simulink model "EdgeImpulse_YOLO_Simulink"  (R2023b)
settings: Solver=FixedStepDiscrete  StartTime=0  StopTime=0.20000000000000001  FixedStep=0.10000000000000001  RelTol=1e-3
InitFcn:
  | ei_sim_prepare('EdgeImpulse_YOLO_Simulink');
model workspace (MAT data in the model file):
  eiBuildInfo.buildKey = 'eb16cb243767a9c4559b'
  eiBuildInfo.height = 180
  eiBuildInfo.width = 180
  eiImageSequence = timeseries
  eiImageSequence.Name = 'unnamed'
  eiImageSequence.DataInfo = tsdata.datametadata
  eiImageSequence.DataInfo.Interpolation = tsdata.interpolation
  eiImageSequence.DataInfo.Interpolation.Fhandle : function handle (value not decoded)
  eiImageSequence.DataInfo.Interpolation.Name = 'zoh'
  eiImageSequence.TimeInfo = tsdata.timemetadata
  eiImageSequence.TimeInfo.Length = 3
  eiImageSequence.TimeInfo.DuplicateTimes = 0
  eiImageSequence.TimeInfo.Time_ = [0; 0.1; 0.2]
  eiImageSequence.TimeInfo.Initialized = 1
  eiImageSequence.QualityInfo = tsdata.qualmetadata
  eiImageSequence.Data_ = [0 0 0 0 0 0 0 0 0 0 0 0 ... (97200 elements, 180x180x3)]
  eiImageSequence.IsTimeFirst_ = 0
  eiNewImageSequence = timeseries
  eiNewImageSequence.Name = 'unnamed'
  eiNewImageSequence.DataInfo = tsdata.datametadata
  eiNewImageSequence.DataInfo.Interpolation = tsdata.interpolation
  eiNewImageSequence.DataInfo.Interpolation.Fhandle : function handle (value not decoded)
  eiNewImageSequence.DataInfo.Interpolation.Name = 'zoh'
  eiNewImageSequence.TimeInfo = tsdata.timemetadata
  eiNewImageSequence.TimeInfo.Length = 3
  eiNewImageSequence.TimeInfo.DuplicateTimes = 0
  eiNewImageSequence.TimeInfo.Time_ = [0; 0.1; 0.2]
  eiNewImageSequence.TimeInfo.Initialized = 1
  eiNewImageSequence.QualityInfo = tsdata.qualmetadata
  eiNewImageSequence.Data_ = [1; 0; 0]
settings Model: Creator=saray  LastModifiedBy=saray
settings SFSimCC: SimCustomInitializer="{ int32_t s=ei_sim_start(5.000000000e-01f,0u,4096u,0u,0); if(s<0) { char e[1024]; ei_get_last_error(e,1024); mexErrMsgIdAndTxt(\"EI:SimInit\",\"%s\",e); } }"  SimCustomTerminator=ei_sim_stop();  SimUserIncludeDirs="\"C:\\Ago-Dic26\\VSCode\\Edge_Impules\\Audrey_Lazara\\EdgeImpulse_MATLAB_Integration\\native\""  SimUserLibraries="\"C:\\Ago-Dic26\\VSCode\\Edge_Impules\\Audrey_Lazara\\EdgeImpulse_MATLAB_Integration\\build\\eb16cb243767a9c4559b\\cmake\\lib\\libei_inference_eb16cb243767a9c4559b.dll.a\""  SimTargetLang=C++
settings SFSimCC: SimCustomHeaderCode=|
  | #include "ei_wrapper.h"
  | #include "mex.h"

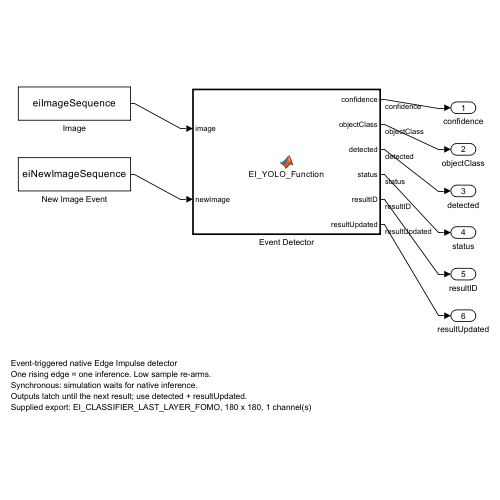
[thumbnail: Simulink's stored preview of the top-level diagram]
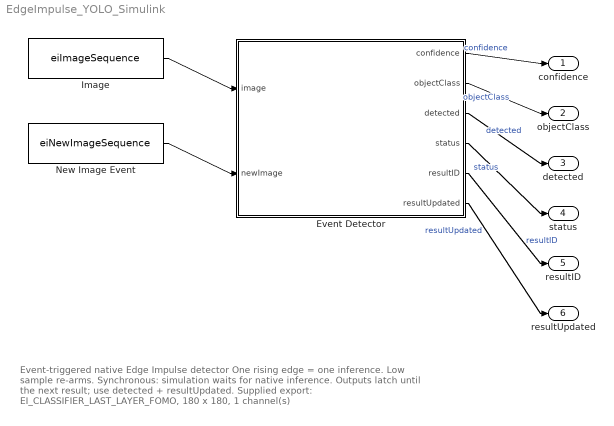
== system EdgeImpulse_YOLO_Simulink ==
  note: Event-triggered native Edge Impulse detector
      | One rising edge = one inference. Low sample re-arms.
      | Synchronous: simulation waits for native inference.
      | Outputs latch until the next result; use detected + resultUpdated.
      | Supplied export: EI_CLASSIFIER_LAST_LAYER_FOMO, 180 x 180, 1 channel(s)
  Event Detector : MATLAB Function  TreatAsAtomicUnit=on
  Image : FromWorkspace  VariableName=eiImageSequence  SampleTime=0.10000000000000001  Interpolate=off  OutputAfterFinalValue=Holding final value
  New Image Event : FromWorkspace  VariableName=eiNewImageSequence  SampleTime=0.10000000000000001  Interpolate=off  OutputAfterFinalValue=Holding final value
  confidence : Outport
  objectClass : Outport  Port=2
  detected : Outport  Port=3
  status : Outport  Port=4
  resultID : Outport  Port=5
  resultUpdated : Outport  Port=6
  wires:
  Image/1 -> Event Detector/1(image)
  New Image Event/1 -> Event Detector/2(newImage)
  Event Detector/1(confidence) -> confidence/1  "confidence"
  Event Detector/2(objectClass) -> objectClass/1  "objectClass"
  Event Detector/3(detected) -> detected/1  "detected"
  Event Detector/4(status) -> status/1  "status"
  Event Detector/5(resultID) -> resultID/1  "resultID"
  Event Detector/6(resultUpdated) -> resultUpdated/1  "resultUpdated"

== matlab function EdgeImpulse_YOLO_Simulink/Event Detector ==
  data: image input uint8 size=[180 180]; confidence output; newImage input boolean size=1; objectClass output; detected output; status output; resultID output; resultUpdated output
function [confidence, objectClass, detected, status, resultID, resultUpdated] = EI_YOLO_Function(image,newImage)
%#codegen
% Rising edges are requests. Keep the full image stable for the source sample.
% A held high signal accepts ONE request. A low sample re-arms the input.
persistent previous heldConfidence heldClass heldDetected heldStatus heldID
if isempty(previous)
    previous=false; heldConfidence=single(0); heldClass=false;
    heldDetected=false; heldStatus=int32(0); heldID=uint64(0);
end
coder.cinclude('ei_wrapper.h');
resultUpdated=false;
if newImage && ~previous
    c=single(0); o=uint8(0); d=uint8(0); id=uint64(0);
    s=int32(0);
    s=coder.ceval('ei_sim_infer',coder.rref(image),uint64(numel(image)), ...
        uint32(size(image,1)),uint32(size(image,2)),coder.wref(c), ...
        coder.wref(o),coder.wref(d),coder.wref(id));
    heldConfidence=c; heldClass=(o~=0); heldDetected=(d~=0);
    heldStatus=s; heldID=id; resultUpdated=true;
end
previous=newImage;
confidence=heldConfidence; objectClass=heldClass; detected=heldDetected;
status=heldStatus; resultID=heldID;
end
